simulink model "lazo"  (R2025b)
settings: Solver=ode4  StartTime=0.0  StopTime=1.5  FixedStep=0.001  RelTol=1e-3
settings Model: Creator=jnune  LastModifiedBy=jnune
settings OptimizationCC: DefaultParameterBehavior=Inlined  EnhancedBackFolding=on  PassReuseOutputArgsAs=Individual arguments  ZeroExternalMemoryAtStartup=off  ZeroInternalMemoryAtStartup=off  MaxStackSize=64  OptimizeBlockOrder=speed  DifferentSizesBufferReuse=on  OptimizationCustomize=off  EfficientTunableParamExpr=on
settings DebuggingCC: ParameterPrecisionLossMsg=none  ParameterTunabilityLossMsg=error
settings HardwareCC: ProdBitPerPointer=32.0  ProdBitPerSizeT=32.0  ProdBitPerPtrDiffT=32.0  ProdLargestAtomicInteger=Long  ProdLargestAtomicFloat=Double  ProdWordSize=32.0  ProdLongLongMode=on  ProdHWDeviceType=ARM Compatible->ARM Cortex-M
settings SFSimCC: MATLABDynamicMemAlloc=off
settings RTWCC: SystemTargetFile=ert.tlc  HardwareBoard=STM32 Nucleo F767ZI  TemplateMakefile=ert_default_tmf  Toolchain=GNU Tools for ARM Embedded Processors  CodeExecutionProfiling=on  CodeProfilingSaveOptions=AllData  Description=Embedded Coder
settings CodeAppCC: ForceParamTrailComments=on  IgnoreCustomStorageClasses=off  OperatorAnnotations=on  SimulinkDataObjDesc=on  SFDataObjDesc=on  InsertBlockDesc=on
settings ERTTargetCC: ExtModeTransport=3.0  ExtModeStaticAlloc=on  ExtModeStaticAllocSize=2000.0  ExtModeMexFile=ext_xcp  ExtModeIntrfLevel=Level2 - Open  TargetLangStandard=C99 (ISO)

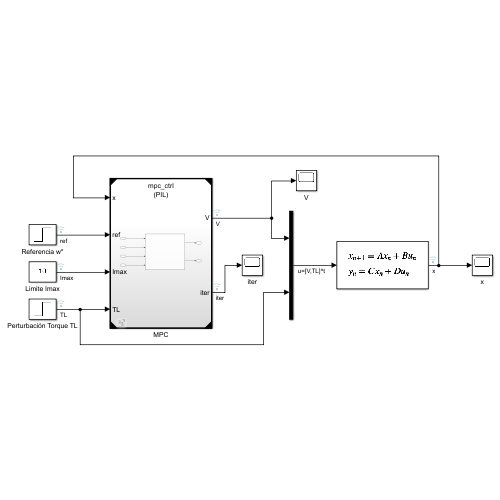
[thumbnail: Simulink's stored preview of the top-level diagram]
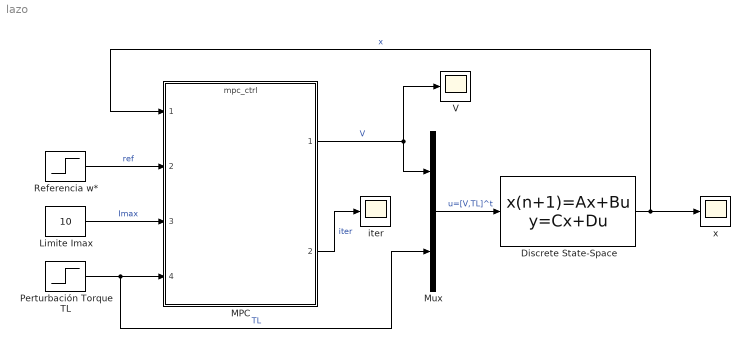
== system lazo ==
  Discrete State-Space : DiscreteStateSpace  A=[0.9802,-1.8840e-04;0.0094,0.9048]  B=[0.0198,9.6101e-05;9.6101e-05,-0.9516]  C=eye(2)  D=zeros(2)  InitialCondition=[0;0]  SampleTime=0.01
  Limite Imax : Constant  Value=10
  MPC : ModelReference  ModelNameDialog=mpc_ctrl  SimulationMode=Processor-in-the-loop (PIL)  ModelReferenceVersion=1.4
  Mux : Mux  Inputs=2
  Perturbación Torque TL : Step  Time=0.8  After=0.005  SampleTime=0.01
  Referencia w* : Step  Time=0.1  SampleTime=0.01
  V : Scope
  iter : Scope
  x : Scope
      settings: ActiveDisplayYMinimum=-27.034704419059068  ActiveDisplayYMaximum=28.381207224274103
  wires:
  Referencia w*/1 -> MPC/2  "ref"
  Limite Imax/1 -> MPC/3  "Imax"
  Perturbación Torque TL/1 -> MPC/4, Mux/2  "TL"
  MPC/1 -> Mux/1, V/1  "V"
  MPC/2 -> iter/1  "iter"
  Mux/1 -> Discrete State-Space/1  "u=[V,TL]^t"
  Discrete State-Space/1 -> x/1, MPC/1  "x"
